simulink model "SZ07_Tekercs"  (R2026a)
settings: Solver=VariableStepAuto  StopTime=800e-3  MaxStep=6e-3/25
libraries: MK_SZ x1
settings Model: Creator=Szalay  LastModifiedBy=Szalay

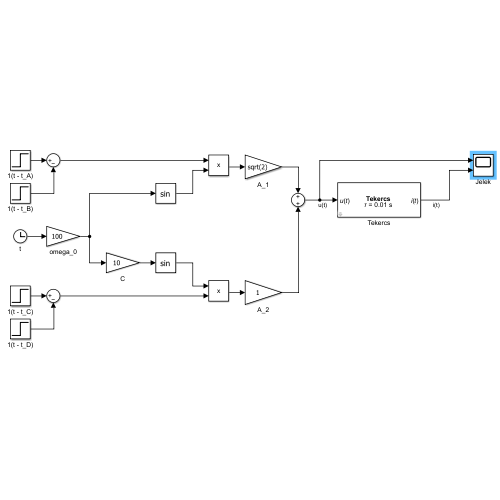
[thumbnail: Simulink's stored preview of the top-level diagram]
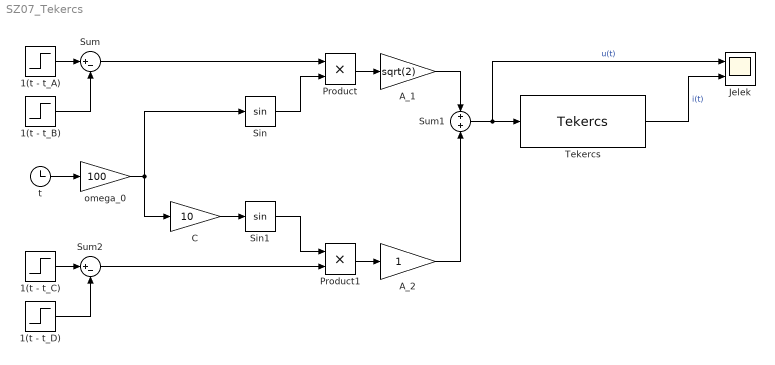
== system SZ07_Tekercs ==
  1(t - t_A) : Step  Time=10e-3  SampleTime=0
  1(t - t_B) : Step  Time=500e-3  SampleTime=0
  1(t - t_C) : Step  Time=600e-3  SampleTime=0
  1(t - t_D) : Step  Time=700e-3  SampleTime=0
  A_1 : Gain  Gain=sqrt(2)
  A_2 : Gain
  C : Gain  Gain=10
  Jelek : Scope  NumInputPorts=2
      settings: ActiveDisplayYMinimum=-1.2525368432297863  ActiveDisplayYMaximum=1.2502780028881071
  Product : Product
  Product1 : Product
  Sin : Trigonometry
  Sin1 : Trigonometry
  Sum : Sum  Inputs=|+-
  Sum1 : Sum  Inputs=+|+
  Sum2 : Sum  Inputs=|+-
  Tekercs : MK_SZ/Tekercs  R=1  L=10e-3  i_0=0
  omega_0 : Gain  Gain=100
  t : Clock
  wires:
  1(t - t_A)/1 -> Sum/1
  1(t - t_B)/1 -> Sum/2
  Sum1/1 -> Jelek/1, Tekercs/1  "u(t)"
  Tekercs/1 -> Jelek/2  "i(t)"
  t/1 -> omega_0/1
  omega_0/1 -> C/1, Sin/1
  Sum/1 -> Product/1
  Sin/1 -> Product/2
  Product/1 -> A_1/1
  A_1/1 -> Sum1/1
  Sum2/1 -> Product1/2
  1(t - t_D)/1 -> Sum2/2
  1(t - t_C)/1 -> Sum2/1
  C/1 -> Sin1/1
  Sin1/1 -> Product1/1
  Product1/1 -> A_2/1
  A_2/1 -> Sum1/2
